simulink model "SmartSense_RD_Linear"  (R2024a)
settings: Solver=FixedStepDiscrete  StartTime=0.0  StopTime=0.0050000000000000001  FixedStep=5.0000000000000004e-06  RelTol=1e-3
settings Model: Creator=DIAW  LastModifiedBy=DIAW

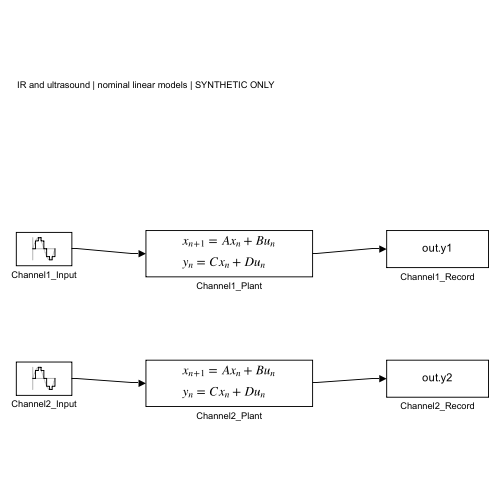
[thumbnail: Simulink's stored preview of the top-level diagram]
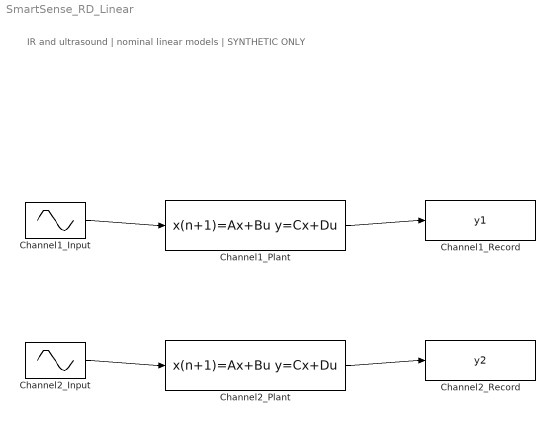
== system SmartSense_RD_Linear ==
  note: IR and ultrasound | nominal linear models | SYNTHETIC ONLY
  Channel1_Input : Sin  Amplitude=9.9999999999999995e-07  Frequency=62831.853071795864  SampleTime=5.0000000000000004e-06
  Channel1_Plant : DiscreteStateSpace  A=[0.002612315967627891 0.007169561617525925 0.0091196590226825525 0.0054738736126996833 0.0026645086743297989 0.00069371496330346944;-0.056062506878132773 -0.14889935408964988 -0.14640846450427888 -0.042391230696712807 -0.011268927087980631 -0.0025727253926748038;0.05197863771582012 0.12645918695131089 0.013433178388338577 -0.41104520319834231 -0.16627765241452699 -0.042007521046019534;0.21217710642648521 0.57666768467521679 0.69425715393796517 0.72610509943534063 -0.11650673210920785 -0.029701704900153281;0.075010636723171265 0.20935045337454217 0.30634636467649456 0.59907835360986295 0.9755489794145229 -0.0062563222189628356;0.0039500317807287253 0.011261174908472747 0.018878397661391808 0.051560875601937645 0.16290520884870169 0.99976032577474605]  B=[-0.00087597666997082468;0.0032486648572387523;0.053044276606621421;0.037505318361585695;0.0079000635614574592;0.00030264451658467914]  C=[0 0 0 0 -130269.3285539121 0]  D=0  SampleTime=5.0000000000000004e-06
  Channel1_Record : ToWorkspace  VariableName=y1  SaveFormat=Timeseries  SampleTime=-1
  Channel2_Input : Sin  Amplitude=0.01  Frequency=251327.41228718346  SampleTime=5.0000000000000004e-06
  Channel2_Plant : DiscreteStateSpace  A=[-0.026199833406930832 0.0082868703428119542 0.093165168452299815 0.072443832099467226 0.026315643022785554 0.0031308187995670402;-0.22912871559266476 -0.4363044460212484 -0.47258015666719577 -0.17105247013137989 -0.045482011177314596 -0.0053698588932081601;0.19649634007640182 0.23713339959180244 -0.016815556052478205 -0.47888247225536701 -0.14819399370305894 -0.017567176547955948;0.3214130916470927 0.6244033165992775 0.80473327665959815 0.74588466731793912 -0.080992770084593227 -0.0096078730761520355;0.087893924818504998 0.19749303346709954 0.34374058337006164 0.61093535514355546 0.98564760661532935 -0.0017031170053928935;0.0009737693558881875 0.0024295663387483408 0.00516467360772427 0.013052608395777121 0.040839773013320757 0.99998573067069407]  B=[-0.00044751702264192352;0.00076756382842344472;0.0025110397784929121;0.001373342575289141;0.00024344233897204687;2.039647828504194e-06]  C=[0 0 0 2416.1188669634676 0 0]  D=0  SampleTime=5.0000000000000004e-06
  Channel2_Record : ToWorkspace  VariableName=y2  SaveFormat=Timeseries  SampleTime=-1
  wires:
  Channel1_Input/1 -> Channel1_Plant/1
  Channel1_Plant/1 -> Channel1_Record/1
  Channel2_Input/1 -> Channel2_Plant/1
  Channel2_Plant/1 -> Channel2_Record/1
